simulink model "gps_transmitter"  (R2025b)
settings: Solver=VariableStepAuto  StartTime=0.0  StopTime=100000  RelTol=1e-3
InitFcn:
  | % 1. Obtener la ruta correcta del archivo .slx usando el comando real
  | modelDir = get_param(bdroot, 'FileName');
  | [projectDir, ~, ~] = fileparts(modelDir);
  | 
  | % 2. Añadir las rutas subiendo un nivel desde Simulink_tests
  | addpath(genpath(fullfile(projectDir, '../src')));
  | addpath(genpath(fullfile(projectDir, '../data')));
settings Model: Creator=User  LastModifiedBy=User

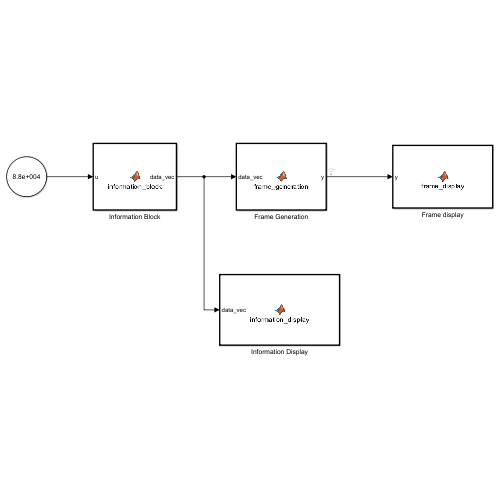
[thumbnail: Simulink's stored preview of the top-level diagram]
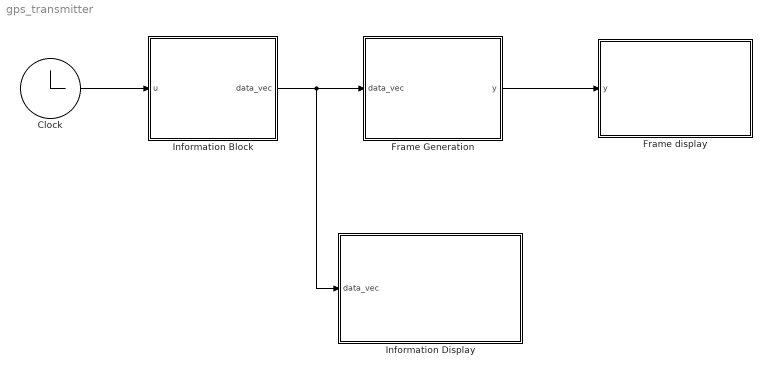
== system gps_transmitter ==
  Clock : Clock
      settings: Decimation=100
  Frame Generation : MATLAB Function  TreatAsAtomicUnit=on
  Frame display : MATLAB Function  TreatAsAtomicUnit=on
  Information Block : MATLAB Function  TreatAsAtomicUnit=on
  Information Display : MATLAB Function  TreatAsAtomicUnit=on
  wires:
  Information Block/1(data_vec) -> Information Display/1(data_vec), Frame Generation/1(data_vec)
  Frame Generation/1(y) -> Frame display/1(y)
  Clock/1 -> Information Block/1(u)

== matlab function gps_transmitter/Information Block ==
  data: u input; data_vec output
function data_vec = information_block(u)
    % 1. Preasignamos el tamaño y tipo exacto (imprescindible en Simulink)
    data_vec = zeros(25, 1); 
    
    % 2. Declaramos la función externa como extrínseca
    coder.extrinsic('pack_orbital_data');
    
    % 3. Llamamos a tu función puente de MATLAB
    data_vec = pack_orbital_data(u);
end

== matlab function gps_transmitter/Frame display ==
  data: y input
function frame_display(y)
    coder.extrinsic('plot_nav_frame');
    plot_nav_frame(y);
end

== matlab function gps_transmitter/Information Display ==
  data: data_vec input
function information_display(data_vec)
%#codegen

coder.extrinsic('gps_information_display');

gps_information_display(data_vec);

end

== matlab function gps_transmitter/Frame Generation ==
  data: data_vec input; y output
function y = frame_generation(data_vec)
    % Predefinir salida (Ajusta el tamaño 50x30 si tu matriz es diferente)
    y = false(50, 30); 
    
    % Declarar extrínsecas si tus funciones internas usan celdas o tipos dinámicos
    coder.extrinsic('gps_icd', 'build_nav_frame');
    
    % 1. Reconstruir el struct mapeando posición por posición
    data = struct();
    data.week      = data_vec(1);
    data.SV_health = data_vec(2);
    data.TGD       = data_vec(3);
    data.IODC      = data_vec(4);
    data.IODE      = data_vec(5);
    data.toc       = data_vec(6);
    data.af2       = data_vec(7);
    data.af1       = data_vec(8);
    data.af0       = data_vec(9);
    data.Crs       = data_vec(10);
    data.Delta_n   = data_vec(11);
    data.M0        = data_vec(12);
    data.Cuc       = data_vec(13);
    data.e         = data_vec(14);
    data.Cus       = data_vec(15);
    data.sqrtA     = data_vec(16);
    data.toe       = data_vec(17);
    data.Cic       = data_vec(18);
    data.Omega0    = data_vec(19);
    data.Cis       = data_vec(20);
    data.i0        = data_vec(21);
    data.Crc       = data_vec(22);
    data.omega     = data_vec(23);
    data.Omega_dot = data_vec(24);
    data.IDOT      = data_vec(25);
    
    % 2. Recuperar parámetros ICD (Estructuras fijas)
    params = gps_icd();
    
    % El tiempo de transmisión (TOW) suele ser el mismo 'toe' o el tiempo actual
    tow_start = data.toe; 
    
    % 3. Llamar a tu script original de generación de subframes
    y = build_nav_frame(data, params, tow_start);
end
